simulink model "HL0905_2"  (R2018b)
settings: Solver=ode3  StartTime=0.0  StopTime=1  FixedStep=0.001  RelTol=1e-3  EnableMultiTasking=on
undefined symbols (not defined in the file): X, Y, Z
libraries: sm_lib x55, nesl_utility x11
(part 1 of 2)
settings Model: Creator=hdu  LastModifiedBy=mails
settings DataIOCC: LimitDataPoints=on  SaveFormat=Array
settings OptimizationCC: LifeSpan=inf
settings DebuggingCC: SolverPrmCheckMsg=warning  SFUnexpectedBacktrackingDiag=warning  SFNoUnconditionalDefaultTransitionDiag=warning  SFExecutionAtInitializationDiag=none
settings HardwareCC: ProdBitPerPointer=32  ProdBitPerSizeT=32  ProdBitPerPtrDiffT=32  ProdLargestAtomicFloat=None  ProdIntDivRoundTo=Undefined  ProdEndianess=Unspecified  ProdWordSize=32  ProdHWDeviceType=32-bit Generic
settings ModelReferenceCC: PropagateSignalLabelsOutOfModel=off
settings SFSimCC: SimUseLocalCustomCode=off
settings RTWCC: RTWUseLocalCustomCode=off
settings CodeAppCC: StateflowObjectComments=on
settings GRTTargetCC: TargetLangStandard=C89/C90 (ANSI)  GeneratePreprocessorConditionals=Disable all
settings ConfigComp: CovMetricSettings=dw  CovHtmlReporting=on  CovSaveCumulativeToWorkspaceVar=on  CovSaveSingleToWorkspaceVar=on  CovExternalEMLEnable=off  CovSFcnEnable=off
settings SimscapeCC: SimscapeNormalizeSystem=off
settings ConfigurationSet: Description=SimMechanics 2G

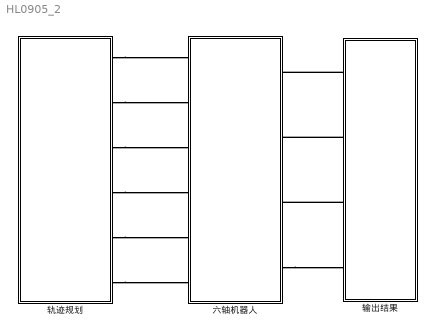
== system HL0905_2 ==
  六轴机器人 : Subsystem
  轨迹规划 : Subsystem
  输出结果 : Subsystem
  connections:
  轨迹规划/RConn1 -- 六轴机器人/LConn1
  轨迹规划/RConn2 -- 六轴机器人/LConn2
  轨迹规划/RConn3 -- 六轴机器人/LConn3
  轨迹规划/RConn4 -- 六轴机器人/LConn4
  轨迹规划/RConn6 -- 六轴机器人/LConn6
  轨迹规划/RConn5 -- 六轴机器人/LConn5
  输出结果/LConn1 -- 六轴机器人/RConn1
  输出结果/LConn2 -- 六轴机器人/RConn2
  输出结果/LConn3 -- 六轴机器人/RConn3
  六轴机器人/RConn4 -- 输出结果/LConn4

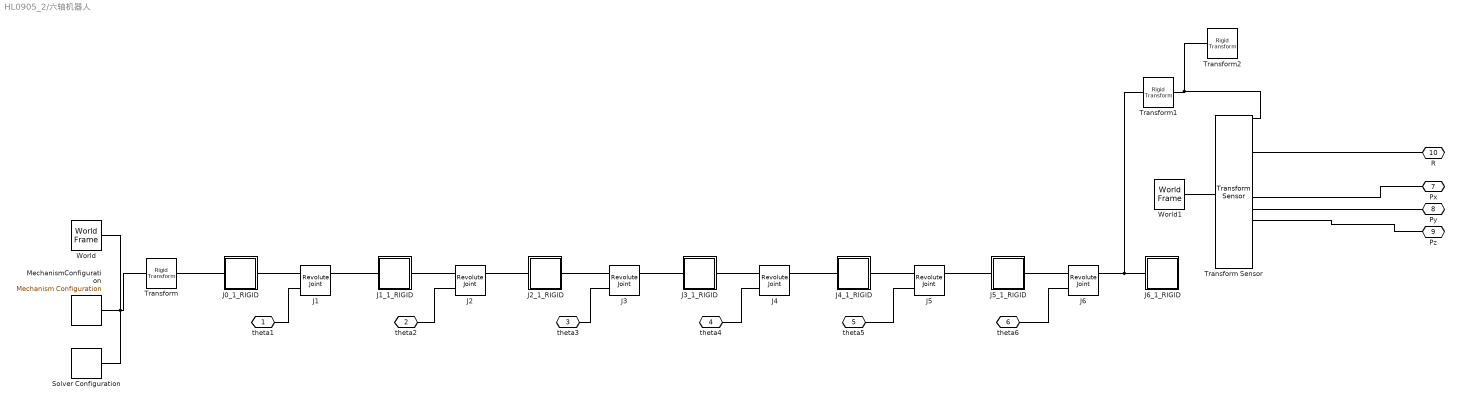
== system HL0905_2/六轴机器人 ==
  J0_1_RIGID : Subsystem
  J1 : sm_lib/Joints/Revolute Joint  SenseConstraintForce=off  SenseConstraintForceX=off  SenseConstraintForceY=off  SenseConstraintForceZ=off  SenseConstraintTorque=off  SenseConstraintTorqueX=off  SenseConstraintTorqueY=off  SenseConstraintTorqueZ=off  SenseTotalForce=off  SenseTotalForceX=off  SenseTotalForceY=off  SenseTotalForceZ=off  SenseTotalTorque=off  SenseTotalTorqueX=off  SenseTotalTorqueY=off  SenseTotalTorqueZ=off  CompositeWrenchDir=FollowerOnBase  CompositeWrenchFrame=BaseFrame  EquilibriumPosition=0  EquilibriumPositionUnits=rad  SpringStiffness=0  SpringStiffnessUnits=m*N/rad  DampingCoefficient=0  DampingCoefficientUnits=m*s*N/rad  TorqueActuationMode=ComputedTorque  MotionActuationMode=InputMotion  SensePosition=off  SenseVelocity=off  SenseAcceleration=off  SenseTorqueForce=on  PositionTargetSpecify=on  PositionTargetPriority=Low  PositionTargetValue=0  PositionTargetValueUnits=deg  VelocityTargetSpecify=off  VelocityTargetPriority=High  VelocityTargetValue=0  VelocityTargetValueUnits=deg/s
  J1_1_RIGID : Subsystem
  J2 : sm_lib/Joints/Revolute Joint  SenseConstraintForce=off  SenseConstraintForceX=off  SenseConstraintForceY=off  SenseConstraintForceZ=off  SenseConstraintTorque=off  SenseConstraintTorqueX=off  SenseConstraintTorqueY=off  SenseConstraintTorqueZ=off  SenseTotalForce=off  SenseTotalForceX=off  SenseTotalForceY=off  SenseTotalForceZ=off  SenseTotalTorque=off  SenseTotalTorqueX=off  SenseTotalTorqueY=off  SenseTotalTorqueZ=off  CompositeWrenchDir=FollowerOnBase  CompositeWrenchFrame=BaseFrame  EquilibriumPosition=0  EquilibriumPositionUnits=rad  SpringStiffness=0  SpringStiffnessUnits=m*N/rad  DampingCoefficient=0  DampingCoefficientUnits=m*s*N/rad  TorqueActuationMode=ComputedTorque  MotionActuationMode=InputMotion  SensePosition=off  SenseVelocity=off  SenseAcceleration=off  SenseTorqueForce=on  PositionTargetSpecify=on  PositionTargetPriority=Low  PositionTargetValue=-6.9319358640751347e-13  PositionTargetValueUnits=deg  VelocityTargetSpecify=off  VelocityTargetPriority=High  VelocityTargetValue=0  VelocityTargetValueUnits=deg/s
  J2_1_RIGID : Subsystem
  J3 : sm_lib/Joints/Revolute Joint  SenseConstraintForce=off  SenseConstraintForceX=off  SenseConstraintForceY=off  SenseConstraintForceZ=off  SenseConstraintTorque=off  SenseConstraintTorqueX=off  SenseConstraintTorqueY=off  SenseConstraintTorqueZ=off  SenseTotalForce=off  SenseTotalForceX=off  SenseTotalForceY=off  SenseTotalForceZ=off  SenseTotalTorque=off  SenseTotalTorqueX=off  SenseTotalTorqueY=off  SenseTotalTorqueZ=off  CompositeWrenchDir=FollowerOnBase  CompositeWrenchFrame=BaseFrame  EquilibriumPosition=0  EquilibriumPositionUnits=rad  SpringStiffness=0  SpringStiffnessUnits=m*N/rad  DampingCoefficient=0  DampingCoefficientUnits=m*s*N/rad  TorqueActuationMode=ComputedTorque  MotionActuationMode=InputMotion  SensePosition=off  SenseVelocity=off  SenseAcceleration=off  SenseTorqueForce=on  PositionTargetSpecify=on  PositionTargetPriority=Low  PositionTargetValue=-90  PositionTargetValueUnits=deg  VelocityTargetSpecify=off  VelocityTargetPriority=High  VelocityTargetValue=0  VelocityTargetValueUnits=deg/s
  J3_1_RIGID : Subsystem
  J4 : sm_lib/Joints/Revolute Joint  SenseConstraintForce=off  SenseConstraintForceX=off  SenseConstraintForceY=off  SenseConstraintForceZ=off  SenseConstraintTorque=off  SenseConstraintTorqueX=off  SenseConstraintTorqueY=off  SenseConstraintTorqueZ=off  SenseTotalForce=off  SenseTotalForceX=off  SenseTotalForceY=off  SenseTotalForceZ=off  SenseTotalTorque=off  SenseTotalTorqueX=off  SenseTotalTorqueY=off  SenseTotalTorqueZ=off  CompositeWrenchDir=FollowerOnBase  CompositeWrenchFrame=BaseFrame  EquilibriumPosition=0  EquilibriumPositionUnits=rad  SpringStiffness=0  SpringStiffnessUnits=m*N/rad  DampingCoefficient=0  DampingCoefficientUnits=m*s*N/rad  TorqueActuationMode=ComputedTorque  MotionActuationMode=InputMotion  SensePosition=off  SenseVelocity=off  SenseAcceleration=off  SenseTorqueForce=on  PositionTargetSpecify=on  PositionTargetPriority=Low  PositionTargetValue=0  PositionTargetValueUnits=deg  VelocityTargetSpecify=off  VelocityTargetPriority=High  VelocityTargetValue=0  VelocityTargetValueUnits=deg/s
  J4_1_RIGID : Subsystem
  J5 : sm_lib/Joints/Revolute Joint  SenseConstraintForce=off  SenseConstraintForceX=off  SenseConstraintForceY=off  SenseConstraintForceZ=off  SenseConstraintTorque=off  SenseConstraintTorqueX=off  SenseConstraintTorqueY=off  SenseConstraintTorqueZ=off  SenseTotalForce=off  SenseTotalForceX=off  SenseTotalForceY=off  SenseTotalForceZ=off  SenseTotalTorque=off  SenseTotalTorqueX=off  SenseTotalTorqueY=off  SenseTotalTorqueZ=off  CompositeWrenchDir=FollowerOnBase  CompositeWrenchFrame=BaseFrame  EquilibriumPosition=0  EquilibriumPositionUnits=rad  SpringStiffness=0  SpringStiffnessUnits=m*N/rad  DampingCoefficient=0  DampingCoefficientUnits=m*s*N/rad  TorqueActuationMode=ComputedTorque  MotionActuationMode=InputMotion  SensePosition=off  SenseVelocity=off  SenseAcceleration=off  SenseTorqueForce=on  PositionTargetSpecify=on  PositionTargetPriority=Low  PositionTargetValue=-4.4527765540484154e-14  PositionTargetValueUnits=deg  VelocityTargetSpecify=off  VelocityTargetPriority=High  VelocityTargetValue=0  VelocityTargetValueUnits=deg/s
  J5_1_RIGID : Subsystem
  J6 : sm_lib/Joints/Revolute Joint  SenseConstraintForce=off  SenseConstraintForceX=off  SenseConstraintForceY=off  SenseConstraintForceZ=off  SenseConstraintTorque=off  SenseConstraintTorqueX=off  SenseConstraintTorqueY=off  SenseConstraintTorqueZ=off  SenseTotalForce=off  SenseTotalForceX=off  SenseTotalForceY=off  SenseTotalForceZ=off  SenseTotalTorque=off  SenseTotalTorqueX=off  SenseTotalTorqueY=off  SenseTotalTorqueZ=off  CompositeWrenchDir=FollowerOnBase  CompositeWrenchFrame=BaseFrame  EquilibriumPosition=0  EquilibriumPositionUnits=rad  SpringStiffness=0  SpringStiffnessUnits=m*N/rad  DampingCoefficient=0  DampingCoefficientUnits=m*s*N/rad  TorqueActuationMode=ComputedTorque  MotionActuationMode=InputMotion  SensePosition=off  SenseVelocity=off  SenseAcceleration=off  SenseTorqueForce=on  PositionTargetSpecify=on  PositionTargetPriority=Low  PositionTargetValue=0  PositionTargetValueUnits=deg  VelocityTargetSpecify=off  VelocityTargetPriority=High  VelocityTargetValue=0  VelocityTargetValueUnits=deg/s
  J6_1_RIGID : Subsystem
  MechanismConfiguration : sm_lib/Utilities/Mechanism Configuration  UniformGravity=Constant  GravityVector=[0 0 -9.81]  GravityUnits=m/s^2  LinearizationDelta=0.001
  Solver Configuration : nesl_utility/Solver Configuration  PhysicalDomain=network_engine_domain  SubClassName=solver  LeftPortType=input  RightPortType=generic  Tones=[]  Harmonics=[]  SimulateNoise=off  Profile=off  UseLocalSampling=off  EnableSwitchedLinearOptims=on  FrequencyDomain=off  UseCCode=off  RelTol=0.001  AbsTol=1e-06  MinStep=1e-09  ToWorkspace=off  RevertToSquareIcSolve=off  NumHomotopyIterations=100  PhasorMode=off  PhasorModeNumHarmonics=1  DoDC=off  ResidualTolerance=1e-09  UseLocalSolver=off  LocalSolverChoice=NE_BACKWARD_EULER_ADVANCER  LocalSolverSampleTime=0.001  DoFixedCost=off  MaxNonlinIter=3  MaxModeIter=2  LinearAlgebra=Sparse  EquationFormulation=NE_TIME_EF  DelaysMemoryBudget=1024  AutomaticFiltering=on  FilteringTimeConstant=0.001  PartitionStorageMethod=AS_NEEDED  PartitionMemoryBudget=1024
  Transform : sm_lib/Frames and Transforms/Rigid Transform  TranslationMethod=Cartesian  TranslationStandardOffset=0  TranslationLengthUnit=mm  TranslationStandardAxis=+Z  TranslationCartesianOffset=[0 0 300]  TranslationROffset=0  TranslationROffsetUnits=m  TranslationZOffset=0  TranslationZOffsetUnits=m  TranslationThetaOffset=0  TranslationThetaOffsetUnits=deg  RotationMethod=ArbitraryAxis  RotationAngleUnits=rad  RotationStandardAxis=+Z  RotationAngle=1.5707963267948966  RotationArbitraryAxis=[7.8504622934188758e-17 -1.2449156633998499e-16 1]  FollAlignAxisA=+X  BaseAlignAxisA=+Y  FollAlignAxisB=+Y  BaseAlignAxisB=+Z  RotationSequenceAxes=FollowerAxes  RotationSequence=XYX  RotationSequenceAngles=[0 0 0]  RotationSequenceAnglesUnits=deg  RotationMatrix=[1 0 0; 0 1 0; 0 0 1]
  Transform Sensor : sm_lib/Frames and Transforms/Transform Sensor  MeasurementFrame=World  SenseAngle=on  SenseAxis=on  SenseAngle1=off  SenseAngle2=off  SenseAngle3=off  SenseQ=off  SenseR=on  SenseOmegaX=on  SenseOmegaY=on  SenseOmegaZ=on  SenseOmega1=off  SenseOmega2=off  SenseOmega3=off  SenseQDot=off  SenseRDot=off  SenseAlphaX=off  SenseAlphaY=off  SenseAlphaZ=off  SenseAlpha1=off  SenseAlpha2=off  SenseAlpha3=off  SenseQDDot=off  SenseRDDot=off  SenseX=on  SenseY=on  SenseZ=on  SenseRad=off  SenseAzim=off  SenseDist=off  SenseInc=off  SenseXDot=off  SenseYDot=on  SenseZDot=on  SenseRadDot=off  SenseAzimDot=off  SenseDistDot=off  SenseIncDot=off  SenseXDDot=off  SenseYDDot=on  SenseZDDot=on  SenseRadDDot=off  SenseAzimDDot=off  SenseDistDDot=off  SenseIncDDot=off
  Transform1 : sm_lib/Frames and Transforms/Rigid Transform  TranslationMethod=Cartesian  TranslationStandardOffset=0  TranslationLengthUnit=mm  TranslationStandardAxis=+X  TranslationCartesianOffset=[0 0 151.194984090458]  TranslationROffset=0  TranslationROffsetUnits=m  TranslationZOffset=0  TranslationZOffsetUnits=m  TranslationThetaOffset=0  TranslationThetaOffsetUnits=deg  RotationMethod=None  RotationAngleUnits=rad  RotationStandardAxis=+Z  RotationAngle=3.1415926535897931  RotationArbitraryAxis=[0 5.5511151231257827e-17 -1]  FollAlignAxisA=+X  BaseAlignAxisA=+Y  FollAlignAxisB=+Y  BaseAlignAxisB=+Z  RotationSequenceAxes=FollowerAxes  RotationSequence=XYX  RotationSequenceAngles=[0 0 0]  RotationSequenceAnglesUnits=deg  RotationMatrix=[1 0 0; 0 1 0; 0 0 1]
  Transform2 : sm_lib/Frames and Transforms/Rigid Transform  TranslationMethod=Cartesian  TranslationStandardOffset=0  TranslationLengthUnit=mm  TranslationStandardAxis=+X  TranslationCartesianOffset=[0 0 124.08]  TranslationROffset=0  TranslationROffsetUnits=m  TranslationZOffset=0  TranslationZOffsetUnits=m  TranslationThetaOffset=0  TranslationThetaOffsetUnits=deg  RotationMethod=None  RotationAngleUnits=rad  RotationStandardAxis=+Z  RotationAngle=3.1415926535897931  RotationArbitraryAxis=[0 5.5511151231257827e-17 -1]  FollAlignAxisA=+X  BaseAlignAxisA=+Y  FollAlignAxisB=+Y  BaseAlignAxisB=+Z  RotationSequenceAxes=FollowerAxes  RotationSequence=XYX  RotationSequenceAngles=[0 0 0]  RotationSequenceAnglesUnits=deg  RotationMatrix=[1 0 0; 0 1 0; 0 0 1]
  World : sm_lib/Frames and Transforms/World Frame
  World1 : sm_lib/Frames and Transforms/World Frame
  theta1 : PMIOPort  Side=Left
  theta2 : PMIOPort  Port=2  Side=Left
  theta3 : PMIOPort  Port=3  Side=Left
  theta4 : PMIOPort  Port=4  Side=Left
  theta5 : PMIOPort  Port=5  Side=Left
  theta6 : PMIOPort  Port=6  Side=Left
  Px : PMIOPort  Port=7  Side=Right
  Py : PMIOPort  Port=8  Side=Right
  Pz : PMIOPort  Port=9  Side=Right
  R : PMIOPort  Port=10  Side=Right
  connections:
  theta3/RConn1 -- J3/LConn2
  theta5/RConn1 -- J5/LConn2
  J0_1_RIGID/LConn1 -- Transform/RConn1
  J4_1_RIGID/LConn1 -- J4/RConn1
  J1_1_RIGID/RConn1 -- J2/LConn1
  J1_1_RIGID/LConn1 -- J1/RConn1
  J6_1_RIGID/LConn1 -- Transform1/LConn1 -- J6/RConn1
  J4_1_RIGID/RConn1 -- J5/LConn1
  J5_1_RIGID/RConn1 -- J6/LConn1
  J2_1_RIGID/LConn1 -- J2/RConn1
  J3_1_RIGID/RConn1 -- J4/LConn1
  J3_1_RIGID/LConn1 -- J3/RConn1
  theta2/RConn1 -- J2/LConn2
  theta6/RConn1 -- J6/LConn2
  theta1/RConn1 -- J1/LConn2
  Transform/LConn1 -- MechanismConfiguration/RConn1 -- Solver Configuration/RConn1 -- World/RConn1
  J0_1_RIGID/RConn1 -- J1/LConn1
  J2_1_RIGID/RConn1 -- J3/LConn1
  J5_1_RIGID/LConn1 -- J5/RConn1
  theta4/RConn1 -- J4/LConn2
  World1/RConn1 -- Transform Sensor/LConn1
  Transform Sensor/RConn8 -- Px/RConn1
  Pz/RConn1 -- Transform Sensor/RConn10
  Transform1/RConn1 -- Transform Sensor/RConn1 -- Transform2/LConn1
  Py/RConn1 -- Transform Sensor/RConn9
  R/RConn1 -- Transform Sensor/RConn4

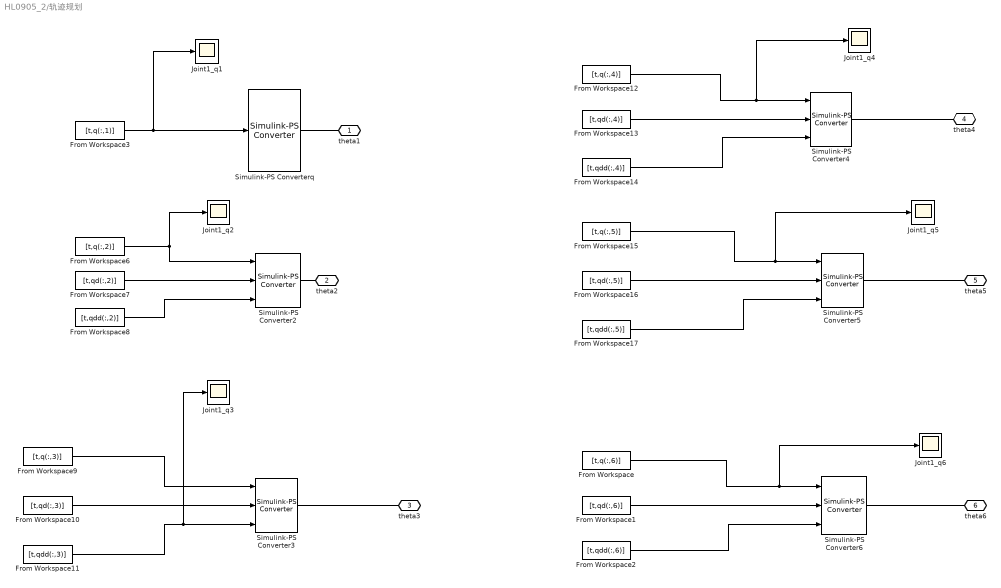
== system HL0905_2/轨迹规划 ==
  From Workspace : FromWorkspace  VariableName=[t,q(:,6)]  SampleTime=0
  From Workspace1 : FromWorkspace  VariableName=[t,qd(:,6)]  SampleTime=0
  From Workspace10 : FromWorkspace  VariableName=[t,qd(:,3)]  SampleTime=0
  From Workspace11 : FromWorkspace  VariableName=[t,qdd(:,3)]  SampleTime=0
  From Workspace12 : FromWorkspace  VariableName=[t,q(:,4)]  SampleTime=0
  From Workspace13 : FromWorkspace  VariableName=[t,qd(:,4)]  SampleTime=0
  From Workspace14 : FromWorkspace  VariableName=[t,qdd(:,4)]  SampleTime=0
  From Workspace15 : FromWorkspace  VariableName=[t,q(:,5)]  SampleTime=0
  From Workspace16 : FromWorkspace  VariableName=[t,qd(:,5)]  SampleTime=0
  From Workspace17 : FromWorkspace  VariableName=[t,qdd(:,5)]  SampleTime=0
  From Workspace2 : FromWorkspace  VariableName=[t,qdd(:,6)]  SampleTime=0
  From Workspace3 : FromWorkspace  VariableName=[t,q(:,1)]  SampleTime=0
  From Workspace6 : FromWorkspace  VariableName=[t,q(:,2)]  SampleTime=0
  From Workspace7 : FromWorkspace  VariableName=[t,qd(:,2)]  SampleTime=0
  From Workspace8 : FromWorkspace  VariableName=[t,qdd(:,2)]  SampleTime=0
  From Workspace9 : FromWorkspace  VariableName=[t,q(:,3)]  SampleTime=0
  Joint1_q{1..6} (6 alike) : Scope
  Simulink-PS Converter{2..6} (5 alike) : nesl_utility/Simulink-PS Converter  PhysicalDomain=network_engine_domain  SubClassName=ps_input  LeftPortType=input  RightPortType=output  PseudoPeriodic=off  Frequencies=[]  NoiseDistribution=none  NoiseParameters=[]  Unit=rad  AffineConversion=off  FilteringAndDerivatives=provide  SimscapeFilterOrder=2  InputFilterTimeConstant=0.01  UdotUserProvided=2
  Simulink-PS Converterq : nesl_utility/Simulink-PS Converter  PhysicalDomain=network_engine_domain  SubClassName=ps_input  LeftPortType=input  RightPortType=output  PseudoPeriodic=off  Frequencies=[]  NoiseDistribution=none  NoiseParameters=[]  Unit=rad  AffineConversion=off  FilteringAndDerivatives=provide  SimscapeFilterOrder=2  InputFilterTimeConstant=0.01  UdotUserProvided=0
  theta1 : PMIOPort  Side=Right
  theta2 : PMIOPort  Port=2  Side=Right
  theta3 : PMIOPort  Port=3  Side=Right
  theta4 : PMIOPort  Port=4  Side=Right
  theta5 : PMIOPort  Port=5  Side=Right
  theta6 : PMIOPort  Port=6  Side=Right
  wires:
  From Workspace1/1 -> Simulink-PS Converter6/2
  From Workspace2/1 -> Simulink-PS Converter6/3
  From Workspace/1 -> Joint1_q6/1, Simulink-PS Converter6/1
  From Workspace3/1 -> Joint1_q1/1, Simulink-PS Converterq/1
  From Workspace7/1 -> Simulink-PS Converter2/2
  From Workspace8/1 -> Simulink-PS Converter2/3
  From Workspace6/1 -> Simulink-PS Converter2/1, Joint1_q2/1
  From Workspace10/1 -> Simulink-PS Converter3/2
  From Workspace11/1 -> Joint1_q3/1, Simulink-PS Converter3/3
  From Workspace9/1 -> Simulink-PS Converter3/1
  From Workspace13/1 -> Simulink-PS Converter4/2
  From Workspace14/1 -> Simulink-PS Converter4/3
  From Workspace12/1 -> Joint1_q4/1, Simulink-PS Converter4/1
  From Workspace16/1 -> Simulink-PS Converter5/2
  From Workspace17/1 -> Simulink-PS Converter5/3
  From Workspace15/1 -> Joint1_q5/1, Simulink-PS Converter5/1
  connections:
  Simulink-PS Converterq/RConn1 -- theta1/RConn1
  Simulink-PS Converter2/RConn1 -- theta2/RConn1
  Simulink-PS Converter3/RConn1 -- theta3/RConn1
  Simulink-PS Converter4/RConn1 -- theta4/RConn1
  Simulink-PS Converter5/RConn1 -- theta5/RConn1
  theta6/RConn1 -- Simulink-PS Converter6/RConn1

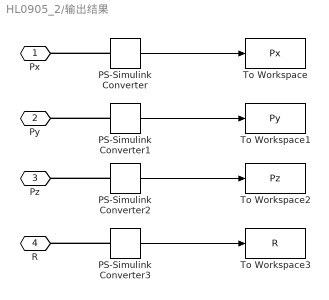
== system HL0905_2/输出结果 ==
  PS-Simulink Converter : nesl_utility/PS-Simulink Converter  PhysicalDomain=network_engine_domain  SubClassName=ps_output  LeftPortType=input  RightPortType=output  PseudoPeriodic=off  Frequencies=[]  Unit=mm  AffineConversion=off
  PS-Simulink Converter1 : nesl_utility/PS-Simulink Converter  PhysicalDomain=network_engine_domain  SubClassName=ps_output  LeftPortType=input  RightPortType=output  PseudoPeriodic=off  Frequencies=[]  Unit=mm  AffineConversion=off
  PS-Simulink Converter2 : nesl_utility/PS-Simulink Converter  PhysicalDomain=network_engine_domain  SubClassName=ps_output  LeftPortType=input  RightPortType=output  PseudoPeriodic=off  Frequencies=[]  Unit=mm  AffineConversion=off
  PS-Simulink Converter3 : nesl_utility/PS-Simulink Converter  PhysicalDomain=network_engine_domain  SubClassName=ps_output  LeftPortType=input  RightPortType=output  PseudoPeriodic=off  Frequencies=[]  Unit=1  AffineConversion=off
  To Workspace : ToWorkspace  VariableName=Px  SampleTime=-1
      settings: Save2DSignal=2-D array (concatenate along first dimension)
  To Workspace1 : ToWorkspace  VariableName=Py  SampleTime=-1
      settings: Save2DSignal=2-D array (concatenate along first dimension)
  To Workspace2 : ToWorkspace  VariableName=Pz  SampleTime=-1
      settings: Save2DSignal=2-D array (concatenate along first dimension)
  To Workspace3 : ToWorkspace  VariableName=R  SampleTime=-1
      settings: Save2DSignal=2-D array (concatenate along first dimension)
  Px : PMIOPort  Side=Left
  Py : PMIOPort  Port=2  Side=Left
  Pz : PMIOPort  Port=3  Side=Left
  R : PMIOPort  Port=4  Side=Left
  wires:
  PS-Simulink Converter/1 -> To Workspace/1
  PS-Simulink Converter1/1 -> To Workspace1/1
  PS-Simulink Converter2/1 -> To Workspace2/1
  PS-Simulink Converter3/1 -> To Workspace3/1
  connections:
  PS-Simulink Converter1/LConn1 -- Py/RConn1
  PS-Simulink Converter/LConn1 -- Px/RConn1
  PS-Simulink Converter2/LConn1 -- Pz/RConn1
  PS-Simulink Converter3/LConn1 -- R/RConn1

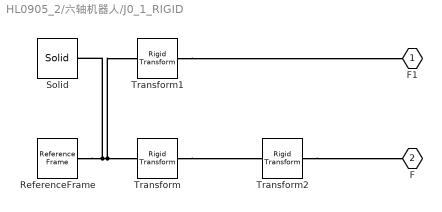
== system HL0905_2/六轴机器人/J0_1_RIGID ==
  ReferenceFrame : sm_lib/Frames and Transforms/Reference Frame
  Solid : sm_lib/Body Elements/Solid  InertiaType=Custom  Mass=7.6540594351842266  MassUnits=kg  CenterOfMass=[22.860239072093147 -147.21867176219041 -1.2431125209809186]  CenterOfMassUnits=mm  MomentsOfInertia=[130694.70688402398 123509.99199142594 133535.69433842544]  MomentsOfInertiaUnits=kg*mm^2  ProductsOfInertia=[-1577.6165993481045 1190.9909643824089 5823.7333434025841]  ProductsOfInertiaUnits=kg*mm^2  BasedOnType=Density  Density=1000  DensityUnits=kg/(m^3)  DoExposeReferenceFrame=on  SerializedFrames=<Frames/>  GraphicType=FromGeometry  MarkerShape=Sphere  MarkerSize=10  MarkerSizeUnits=m  GraphicVisPropType=SimpleVisualProperties  GraphicDiffuseColor=[0.2 0.2 0.2]  GraphicSpecularColor=[0.5 0.5 0.5 1.0]  GraphicAmbientColor=[0.15 0.15 0.15 1.0]  GraphicEmissiveColor=[0.0 0.0 0.0 1.0]  GraphicShininess=75  GraphicOpacity=1  GeometryShape=FromFile  RectangleSize=[1 1]  RectangleSizeUnits=m  BrickDimensions=[1 1 1]  BrickDimensionUnits=m  CylinderRadius=1  CylinderRadiusUnits=m  CylinderLength=1  CylinderLengthUnits=m  SphereRadius=1  SphereRadiusUnits=m  EllipsoidRadii=[1 1 1]  EllipsoidRadiiUnits=m  ExtrusionCrossSection=[1 1; -1 1; -1 -1; 1 -1]  ExtrusionCrossSectionUnits=m  ExtrusionLength=1  ExtrusionLengthUnits=m  PolygonNumSides=3  PolygonOuterRadius=1  PolygonOuterRadiusUnits=m  ExtGeomFileType=STL  ExtGeomFileName=J0_默认_sldprt.STL  ExtGeomFileUnits=mm  RevolutionCrossSection=[1 1; 1 -1; 2 -1; 2 1]  RevolutionCrossSectionUnits=m  RevolutionExtent=Full  RevolutionAngle=180  RevolutionAngleUnits=deg
  Transform : sm_lib/Frames and Transforms/Rigid Transform  TranslationMethod=Cartesian  TranslationStandardOffset=0  TranslationLengthUnit=mm  TranslationStandardAxis=+Z  TranslationCartesianOffset=[-1.1006414838582221e-13 -330.45657177129794 1.4155343563970754e-12]  TranslationROffset=0  TranslationROffsetUnits=m  TranslationZOffset=0  TranslationZOffsetUnits=m  TranslationThetaOffset=0  TranslationThetaOffsetUnits=deg  RotationMethod=ArbitraryAxis  RotationAngleUnits=rad  RotationStandardAxis=+Z  RotationAngle=2.0943951023931957  RotationArbitraryAxis=[-0.57735026918962584 -0.57735026918962562 -0.57735026918962584]  FollAlignAxisA=+X  BaseAlignAxisA=+Y  FollAlignAxisB=+Y  BaseAlignAxisB=+Z  RotationSequenceAxes=FollowerAxes  RotationSequence=XYX  RotationSequenceAngles=[0 0 0]  RotationSequenceAnglesUnits=deg  RotationMatrix=[1 0 0; 0 1 0; 0 0 1]
  Transform1 : sm_lib/Frames and Transforms/Rigid Transform  TranslationMethod=Cartesian  TranslationStandardOffset=0  TranslationLengthUnit=mm  TranslationStandardAxis=+Z  TranslationCartesianOffset=[0 0 0]  TranslationROffset=0  TranslationROffsetUnits=m  TranslationZOffset=0  TranslationZOffsetUnits=m  TranslationThetaOffset=0  TranslationThetaOffsetUnits=deg  RotationMethod=ArbitraryAxis  RotationAngleUnits=rad  RotationStandardAxis=+Z  RotationAngle=2.0943951023931957  RotationArbitraryAxis=[-0.57735026918962584 -0.57735026918962562 -0.57735026918962584]  FollAlignAxisA=+X  BaseAlignAxisA=+Y  FollAlignAxisB=+Y  BaseAlignAxisB=+Z  RotationSequenceAxes=FollowerAxes  RotationSequence=XYX  RotationSequenceAngles=[0 0 0]  RotationSequenceAnglesUnits=deg  RotationMatrix=[1 0 0; 0 1 0; 0 0 1]
  Transform2 : sm_lib/Frames and Transforms/Rigid Transform  TranslationMethod=Cartesian  TranslationStandardOffset=0  TranslationLengthUnit=mm  TranslationStandardAxis=+Z  TranslationCartesianOffset=[0 0 0]  TranslationROffset=0  TranslationROffsetUnits=m  TranslationZOffset=0  TranslationZOffsetUnits=m  TranslationThetaOffset=0  TranslationThetaOffsetUnits=deg  RotationMethod=StandardAxis  RotationAngleUnits=deg  RotationStandardAxis=+Z  RotationAngle=-90  RotationArbitraryAxis=[-0.57735026918962584 -0.57735026918962562 -0.57735026918962584]  FollAlignAxisA=+X  BaseAlignAxisA=+Y  FollAlignAxisB=+Y  BaseAlignAxisB=+Z  RotationSequenceAxes=FollowerAxes  RotationSequence=XYX  RotationSequenceAngles=[0 0 0]  RotationSequenceAnglesUnits=deg  RotationMatrix=[1 0 0; 0 1 0; 0 0 1]
  F1 : PMIOPort  Side=Left
  F : PMIOPort  Port=2  Side=Right
  connections:
  Solid/RConn1 -- ReferenceFrame/RConn1 -- Transform/LConn1 -- Transform1/LConn1
  Transform/RConn1 -- Transform2/LConn1
  Transform2/RConn1 -- F/RConn1
  Transform1/RConn1 -- F1/RConn1

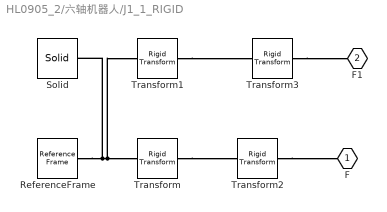
== system HL0905_2/六轴机器人/J1_1_RIGID ==
  ReferenceFrame : sm_lib/Frames and Transforms/Reference Frame
  Solid : sm_lib/Body Elements/Solid  InertiaType=Custom  Mass=10.630000000000001  MassUnits=kg  CenterOfMass=[38.979999999999997 5.6399999999999997 -87]  CenterOfMassUnits=mm  MomentsOfInertia=[58730.529999999999 75050.639999999999 55241.57]  MomentsOfInertiaUnits=kg*mm^2  ProductsOfInertia=[-528.18999999999994 -10070.20999999999 -853.15999999999997]  ProductsOfInertiaUnits=kg*mm^2  BasedOnType=Density  Density=1000  DensityUnits=kg/(m^3)  DoExposeReferenceFrame=on  SerializedFrames=<Frames/>  GraphicType=FromGeometry  MarkerShape=Sphere  MarkerSize=10  MarkerSizeUnits=m  GraphicVisPropType=SimpleVisualProperties  GraphicDiffuseColor=[1 1 1]  GraphicSpecularColor=[0.5 0.5 0.5 1.0]  GraphicAmbientColor=[0.15 0.15 0.15 1.0]  GraphicEmissiveColor=[0.0 0.0 0.0 1.0]  GraphicShininess=75  GraphicOpacity=1  GeometryShape=FromFile  RectangleSize=[1 1]  RectangleSizeUnits=m  BrickDimensions=[1 1 1]  BrickDimensionUnits=m  CylinderRadius=1  CylinderRadiusUnits=m  CylinderLength=1  CylinderLengthUnits=m  SphereRadius=1  SphereRadiusUnits=m  EllipsoidRadii=[1 1 1]  EllipsoidRadiiUnits=m  ExtrusionCrossSection=[1 1; -1 1; -1 -1; 1 -1]  ExtrusionCrossSectionUnits=m  ExtrusionLength=1  ExtrusionLengthUnits=m  PolygonNumSides=3  PolygonOuterRadius=1  PolygonOuterRadiusUnits=m  ExtGeomFileType=STL  ExtGeomFileName=J1_默认_sldprt.STL  ExtGeomFileUnits=mm  RevolutionCrossSection=[1 1; 1 -1; 2 -1; 2 1]  RevolutionCrossSectionUnits=m  RevolutionExtent=Full  RevolutionAngle=180  RevolutionAngleUnits=deg
  Transform : sm_lib/Frames and Transforms/Rigid Transform  TranslationMethod=Cartesian  TranslationStandardOffset=0  TranslationLengthUnit=mm  TranslationStandardAxis=+Z  TranslationCartesianOffset=[-1.5175638523601265e-12 0.46986063114494953 -521.58681036714142]  TranslationROffset=0  TranslationROffsetUnits=m  TranslationZOffset=0  TranslationZOffsetUnits=m  TranslationThetaOffset=0  TranslationThetaOffsetUnits=deg  RotationMethod=ArbitraryAxis  RotationAngleUnits=rad  RotationStandardAxis=+Z  RotationAngle=4.6857050202360969e-15  RotationArbitraryAxis=[0.043683951669101606 0.99904540055323376 1.0224735728616534e-16]  FollAlignAxisA=+X  BaseAlignAxisA=+Y  FollAlignAxisB=+Y  BaseAlignAxisB=+Z  RotationSequenceAxes=FollowerAxes  RotationSequence=XYX  RotationSequenceAngles=[0 0 0]  RotationSequenceAnglesUnits=deg  RotationMatrix=[1 0 0; 0 1 0; 0 0 1]
  Transform1 : sm_lib/Frames and Transforms/Rigid Transform  TranslationMethod=Cartesian  TranslationStandardOffset=0  TranslationLengthUnit=mm  TranslationStandardAxis=+Z  TranslationCartesianOffset=[-157.5018651542409 0.46986063114702603 -0.13023859582908526]  TranslationROffset=0  TranslationROffsetUnits=m  TranslationZOffset=0  TranslationZOffsetUnits=m  TranslationThetaOffset=0  TranslationThetaOffsetUnits=deg  RotationMethod=ArbitraryAxis  RotationAngleUnits=rad  RotationStandardAxis=+Z  RotationAngle=2.0943951023932077  RotationArbitraryAxis=[0.57735026918961752 0.57735026918962995 0.57735026918962984]  FollAlignAxisA=+X  BaseAlignAxisA=+Y  FollAlignAxisB=+Y  BaseAlignAxisB=+Z  RotationSequenceAxes=FollowerAxes  RotationSequence=XYX  RotationSequenceAngles=[0 0 0]  RotationSequenceAnglesUnits=deg  RotationMatrix=[1 0 0; 0 1 0; 0 0 1]
  Transform2 : sm_lib/Frames and Transforms/Rigid Transform  TranslationMethod=Cartesian  TranslationStandardOffset=0  TranslationLengthUnit=mm  TranslationStandardAxis=+Z  TranslationCartesianOffset=[0 0 0]  TranslationROffset=0  TranslationROffsetUnits=m  TranslationZOffset=0  TranslationZOffsetUnits=m  TranslationThetaOffset=0  TranslationThetaOffsetUnits=deg  RotationMethod=StandardAxis  RotationAngleUnits=deg  RotationStandardAxis=+Z  RotationAngle=90  RotationArbitraryAxis=[-0.57735026918962584 -0.57735026918962562 -0.57735026918962584]  FollAlignAxisA=+X  BaseAlignAxisA=+Y  FollAlignAxisB=+Y  BaseAlignAxisB=+Z  RotationSequenceAxes=FollowerAxes  RotationSequence=XYX  RotationSequenceAngles=[0 0 0]  RotationSequenceAnglesUnits=deg  RotationMatrix=[1 0 0; 0 1 0; 0 0 1]
  Transform3 : sm_lib/Frames and Transforms/Rigid Transform  TranslationMethod=Cartesian  TranslationStandardOffset=0  TranslationLengthUnit=mm  TranslationStandardAxis=+Z  TranslationCartesianOffset=[0 0 0]  TranslationROffset=0  TranslationROffsetUnits=m  TranslationZOffset=0  TranslationZOffsetUnits=m  TranslationThetaOffset=0  TranslationThetaOffsetUnits=deg  RotationMethod=AlignedAxes  RotationAngleUnits=deg  RotationStandardAxis=+Z  RotationAngle=90  RotationArbitraryAxis=[-0.57735026918962584 -0.57735026918962562 -0.57735026918962584]  FollAlignAxisA=+Z  BaseAlignAxisA=-Z  FollAlignAxisB=+Y  BaseAlignAxisB=+X  RotationSequenceAxes=FollowerAxes  RotationSequence=XYX  RotationSequenceAngles=[0 0 0]  RotationSequenceAnglesUnits=deg  RotationMatrix=[1 0 0; 0 1 0; 0 0 1]
  F : PMIOPort  Side=Left
  F1 : PMIOPort  Port=2  Side=Right
  connections:
  Solid/RConn1 -- ReferenceFrame/RConn1 -- Transform/LConn1 -- Transform1/LConn1
  Transform2/RConn1 -- F/RConn1
  Transform3/RConn1 -- F1/RConn1
  Transform/RConn1 -- Transform2/LConn1
  Transform1/RConn1 -- Transform3/LConn1

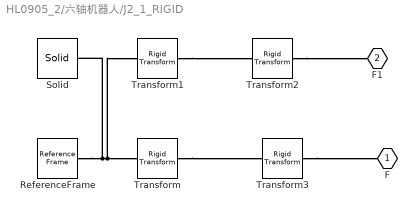
== system HL0905_2/六轴机器人/J2_1_RIGID ==
  ReferenceFrame : sm_lib/Frames and Transforms/Reference Frame
  Solid : sm_lib/Body Elements/Solid  InertiaType=Custom  Mass=13.369999999999999  MassUnits=kg  CenterOfMass=[-9.3499999999999996 -290.32999999999998 13.24]  CenterOfMassUnits=mm  MomentsOfInertia=[305534.1999999999 54660.519999999997 294009.64000000001]  MomentsOfInertiaUnits=kg*mm^2  ProductsOfInertia=[5354.0299999999979 -968.77999999999997 5458.8599999999997]  ProductsOfInertiaUnits=kg*mm^2  BasedOnType=Density  Density=1000  DensityUnits=kg/(m^3)  DoExposeReferenceFrame=on  SerializedFrames=<Frames/>  GraphicType=FromGeometry  MarkerShape=Sphere  MarkerSize=10  MarkerSizeUnits=m  GraphicVisPropType=SimpleVisualProperties  GraphicDiffuseColor=[1 1 1]  GraphicSpecularColor=[0.5 0.5 0.5 1.0]  GraphicAmbientColor=[0.15 0.15 0.15 1.0]  GraphicEmissiveColor=[0.0 0.0 0.0 1.0]  GraphicShininess=75  GraphicOpacity=1  GeometryShape=FromFile  RectangleSize=[1 1]  RectangleSizeUnits=m  BrickDimensions=[1 1 1]  BrickDimensionUnits=m  CylinderRadius=1  CylinderRadiusUnits=m  CylinderLength=1  CylinderLengthUnits=m  SphereRadius=1  SphereRadiusUnits=m  EllipsoidRadii=[1 1 1]  EllipsoidRadiiUnits=m  ExtrusionCrossSection=[1 1; -1 1; -1 -1; 1 -1]  ExtrusionCrossSectionUnits=m  ExtrusionLength=1  ExtrusionLengthUnits=m  PolygonNumSides=3  PolygonOuterRadius=1  PolygonOuterRadiusUnits=m  ExtGeomFileType=STL  ExtGeomFileName=J2_默认_sldprt.STL  ExtGeomFileUnits=mm  RevolutionCrossSection=[1 1; 1 -1; 2 -1; 2 1]  RevolutionCrossSectionUnits=m  RevolutionExtent=Full  RevolutionAngle=180  RevolutionAngleUnits=deg
  Transform : sm_lib/Frames and Transforms/Rigid Transform  TranslationMethod=Cartesian  TranslationStandardOffset=0  TranslationLengthUnit=mm  TranslationStandardAxis=+Z  TranslationCartesianOffset=[-1.1161902030621819e-12 -450.00000000000068 -157.50186515424167]  TranslationROffset=0  TranslationROffsetUnits=m  TranslationZOffset=0  TranslationZOffsetUnits=m  TranslationThetaOffset=0  TranslationThetaOffsetUnits=deg  RotationMethod=ArbitraryAxis  RotationAngleUnits=rad  RotationStandardAxis=+Z  RotationAngle=2.2022005471504983e-14  RotationArbitraryAxis=[-0.2016570245724037 0.97945619832670661 -2.1748296459883953e-15]  FollAlignAxisA=+X  BaseAlignAxisA=+Y  FollAlignAxisB=+Y  BaseAlignAxisB=+Z  RotationSequenceAxes=FollowerAxes  RotationSequence=XYX  RotationSequenceAngles=[0 0 0]  RotationSequenceAnglesUnits=deg  RotationMatrix=[1 0 0; 0 1 0; 0 0 1]
  Transform1 : sm_lib/Frames and Transforms/Rigid Transform  TranslationMethod=Cartesian  TranslationStandardOffset=0  TranslationLengthUnit=mm  TranslationStandardAxis=+Z  TranslationCartesianOffset=[0 0 -249.10747383836633]  TranslationROffset=0  TranslationROffsetUnits=m  TranslationZOffset=0  TranslationZOffsetUnits=m  TranslationThetaOffset=0  TranslationThetaOffsetUnits=deg  RotationMethod=ArbitraryAxis  RotationAngleUnits=rad  RotationStandardAxis=+Z  RotationAngle=0  RotationArbitraryAxis=[0 0 0]  FollAlignAxisA=+X  BaseAlignAxisA=+Y  FollAlignAxisB=+Y  BaseAlignAxisB=+Z  RotationSequenceAxes=FollowerAxes  RotationSequence=XYX  RotationSequenceAngles=[0 0 0]  RotationSequenceAnglesUnits=deg  RotationMatrix=[1 0 0; 0 1 0; 0 0 1]
  Transform2 : sm_lib/Frames and Transforms/Rigid Transform  TranslationMethod=Cartesian  TranslationStandardOffset=0  TranslationLengthUnit=mm  TranslationStandardAxis=+Z  TranslationCartesianOffset=[0 0 0]  TranslationROffset=0  TranslationROffsetUnits=m  TranslationZOffset=0  TranslationZOffsetUnits=m  TranslationThetaOffset=0  TranslationThetaOffsetUnits=deg  RotationMethod=AlignedAxes  RotationAngleUnits=deg  RotationStandardAxis=+Z  RotationAngle=90  RotationArbitraryAxis=[-0.57735026918962584 -0.57735026918962562 -0.57735026918962584]  FollAlignAxisA=+Z  BaseAlignAxisA=-Z  FollAlignAxisB=+Y  BaseAlignAxisB=+X  RotationSequenceAxes=FollowerAxes  RotationSequence=XYX  RotationSequenceAngles=[0 0 0]  RotationSequenceAnglesUnits=deg  RotationMatrix=[1 0 0; 0 1 0; 0 0 1]
  Transform3 : sm_lib/Frames and Transforms/Rigid Transform  TranslationMethod=Cartesian  TranslationStandardOffset=0  TranslationLengthUnit=mm  TranslationStandardAxis=+Z  TranslationCartesianOffset=[0 0 0]  TranslationROffset=0  TranslationROffsetUnits=m  TranslationZOffset=0  TranslationZOffsetUnits=m  TranslationThetaOffset=0  TranslationThetaOffsetUnits=deg  RotationMethod=AlignedAxes  RotationAngleUnits=deg  RotationStandardAxis=+Z  RotationAngle=90  RotationArbitraryAxis=[-0.57735026918962584 -0.57735026918962562 -0.57735026918962584]  FollAlignAxisA=+Z  BaseAlignAxisA=-Z  FollAlignAxisB=+Y  BaseAlignAxisB=+X  RotationSequenceAxes=FollowerAxes  RotationSequence=XYX  RotationSequenceAngles=[0 0 0]  RotationSequenceAnglesUnits=deg  RotationMatrix=[1 0 0; 0 1 0; 0 0 1]
  F : PMIOPort  Side=Left
  F1 : PMIOPort  Port=2  Side=Right
  connections:
  Solid/RConn1 -- ReferenceFrame/RConn1 -- Transform/LConn1 -- Transform1/LConn1
  Transform3/RConn1 -- F/RConn1
  Transform2/RConn1 -- F1/RConn1
  Transform/RConn1 -- Transform3/LConn1
  Transform1/RConn1 -- Transform2/LConn1

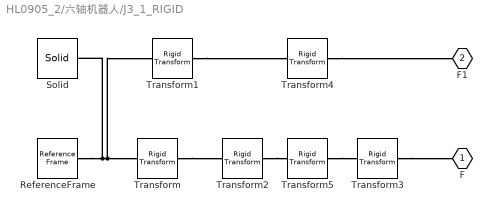
== system HL0905_2/六轴机器人/J3_1_RIGID ==
  ReferenceFrame : sm_lib/Frames and Transforms/Reference Frame
  Solid : sm_lib/Body Elements/Solid  InertiaType=Custom  Mass=5.2930000000000001  MassUnits=kg  CenterOfMass=[82.347999999999999 -6.7000000000000002 -16.399999999999999]  CenterOfMassUnits=mm  MomentsOfInertia=[9712.7630000000008 14300.983 15335.696]  MomentsOfInertiaUnits=kg*mm^2  ProductsOfInertia=[137.73699999999999 1087.2009999999993 296.08499999999998]  ProductsOfInertiaUnits=kg*mm^2  BasedOnType=Density  Density=1000  DensityUnits=kg/(m^3)  DoExposeReferenceFrame=on  SerializedFrames=<Frames/>  GraphicType=FromGeometry  MarkerShape=Sphere  MarkerSize=10  MarkerSizeUnits=m  GraphicVisPropType=SimpleVisualProperties  GraphicDiffuseColor=[1 1 1]  GraphicSpecularColor=[0.5 0.5 0.5 1.0]  GraphicAmbientColor=[0.15 0.15 0.15 1.0]  GraphicEmissiveColor=[0.0 0.0 0.0 1.0]  GraphicShininess=75  GraphicOpacity=1  GeometryShape=FromFile  RectangleSize=[1 1]  RectangleSizeUnits=m  BrickDimensions=[1 1 1]  BrickDimensionUnits=m  CylinderRadius=1  CylinderRadiusUnits=m  CylinderLength=1  CylinderLengthUnits=m  SphereRadius=1  SphereRadiusUnits=m  EllipsoidRadii=[1 1 1]  EllipsoidRadiiUnits=m  ExtrusionCrossSection=[1 1; -1 1; -1 -1; 1 -1]  ExtrusionCrossSectionUnits=m  ExtrusionLength=1  ExtrusionLengthUnits=m  PolygonNumSides=3  PolygonOuterRadius=1  PolygonOuterRadiusUnits=m  ExtGeomFileType=STL  ExtGeomFileName=J3_默认_sldprt.STL  ExtGeomFileUnits=mm  RevolutionCrossSection=[1 1; 1 -1; 2 -1; 2 1]  RevolutionCrossSectionUnits=m  RevolutionExtent=Full  RevolutionAngle=180  RevolutionAngleUnits=deg
  Transform : sm_lib/Frames and Transforms/Rigid Transform  TranslationMethod=Cartesian  TranslationStandardOffset=0  TranslationLengthUnit=mm  TranslationStandardAxis=+Z  TranslationCartesianOffset=[80.000000000010388 -1.3557155398302712e-11 249.10747383836627]  TranslationROffset=0  TranslationROffsetUnits=m  TranslationZOffset=0  TranslationZOffsetUnits=m  TranslationThetaOffset=0  TranslationThetaOffsetUnits=deg  RotationMethod=ArbitraryAxis  RotationAngleUnits=rad  RotationStandardAxis=+Z  RotationAngle=3.1415926535897931  RotationArbitraryAxis=[1 -3.7970713377376732e-47 -7.7524554575046664e-17]  FollAlignAxisA=+X  BaseAlignAxisA=+Y  FollAlignAxisB=+Y  BaseAlignAxisB=+Z  RotationSequenceAxes=FollowerAxes  RotationSequence=XYX  RotationSequenceAngles=[0 0 0]  RotationSequenceAnglesUnits=deg  RotationMatrix=[1 0 0; 0 1 0; 0 0 1]
  Transform1 : sm_lib/Frames and Transforms/Rigid Transform  TranslationMethod=Cartesian  TranslationStandardOffset=0  TranslationLengthUnit=mm  TranslationStandardAxis=+Z  TranslationCartesianOffset=[-61.209572476958321 1.1102230246251565e-13 0]  TranslationROffset=0  TranslationROffsetUnits=m  TranslationZOffset=0  TranslationZOffsetUnits=m  TranslationThetaOffset=0  TranslationThetaOffsetUnits=deg  RotationMethod=ArbitraryAxis  RotationAngleUnits=rad  RotationStandardAxis=+Z  RotationAngle=2.0943951023931957  RotationArbitraryAxis=[0.57735026918962573 0.57735026918962562 0.57735026918962573]  FollAlignAxisA=+X  BaseAlignAxisA=+Y  FollAlignAxisB=+Y  BaseAlignAxisB=+Z  RotationSequenceAxes=FollowerAxes  RotationSequence=XYX  RotationSequenceAngles=[0 0 0]  RotationSequenceAnglesUnits=deg  RotationMatrix=[1 0 0; 0 1 0; 0 0 1]
  Transform2 : sm_lib/Frames and Transforms/Rigid Transform  TranslationMethod=Cartesian  TranslationStandardOffset=0  TranslationLengthUnit=mm  TranslationStandardAxis=+Z  TranslationCartesianOffset=[0 0 0]  TranslationROffset=0  TranslationROffsetUnits=m  TranslationZOffset=0  TranslationZOffsetUnits=m  TranslationThetaOffset=0  TranslationThetaOffsetUnits=deg  RotationMethod=AlignedAxes  RotationAngleUnits=deg  RotationStandardAxis=+Z  RotationAngle=90  RotationArbitraryAxis=[-0.57735026918962584 -0.57735026918962562 -0.57735026918962584]  FollAlignAxisA=+Z  BaseAlignAxisA=-Z  FollAlignAxisB=+Y  BaseAlignAxisB=+X  RotationSequenceAxes=FollowerAxes  RotationSequence=XYX  RotationSequenceAngles=[0 0 0]  RotationSequenceAnglesUnits=deg  RotationMatrix=[1 0 0; 0 1 0; 0 0 1]
  Transform3 : sm_lib/Frames and Transforms/Rigid Transform  TranslationMethod=Cartesian  TranslationStandardOffset=0  TranslationLengthUnit=mm  TranslationStandardAxis=+Z  TranslationCartesianOffset=[0 0 0]  TranslationROffset=0  TranslationROffsetUnits=m  TranslationZOffset=0  TranslationZOffsetUnits=m  TranslationThetaOffset=0  TranslationThetaOffsetUnits=deg  RotationMethod=StandardAxis  RotationAngleUnits=deg  RotationStandardAxis=+Z  RotationAngle=180  RotationArbitraryAxis=[-0.57735026918962584 -0.57735026918962562 -0.57735026918962584]  FollAlignAxisA=+Z  BaseAlignAxisA=-Z  FollAlignAxisB=+Y  BaseAlignAxisB=+X  RotationSequenceAxes=FollowerAxes  RotationSequence=XYX  RotationSequenceAngles=[0 0 0]  RotationSequenceAnglesUnits=deg  RotationMatrix=[1 0 0; 0 1 0; 0 0 1]
  Transform4 : sm_lib/Frames and Transforms/Rigid Transform  TranslationMethod=Cartesian  TranslationStandardOffset=0  TranslationLengthUnit=mm  TranslationStandardAxis=+Z  TranslationCartesianOffset=[0 0 0]  TranslationROffset=0  TranslationROffsetUnits=m  TranslationZOffset=0  TranslationZOffsetUnits=m  TranslationThetaOffset=0  TranslationThetaOffsetUnits=deg  RotationMethod=StandardAxis  RotationAngleUnits=deg  RotationStandardAxis=+X  RotationAngle=180  RotationArbitraryAxis=[-0.57735026918962584 -0.57735026918962562 -0.57735026918962584]  FollAlignAxisA=+Z  BaseAlignAxisA=-Z  FollAlignAxisB=+Y  BaseAlignAxisB=+X  RotationSequenceAxes=FollowerAxes  RotationSequence=XYX  RotationSequenceAngles=[0 0 0]  RotationSequenceAnglesUnits=deg  RotationMatrix=[1 0 0; 0 1 0; 0 0 1]
  Transform5 : sm_lib/Frames and Transforms/Rigid Transform  TranslationMethod=Cartesian  TranslationStandardOffset=0  TranslationLengthUnit=mm  TranslationStandardAxis=+Z  TranslationCartesianOffset=[0 0 0]  TranslationROffset=0  TranslationROffsetUnits=m  TranslationZOffset=0  TranslationZOffsetUnits=m  TranslationThetaOffset=0  TranslationThetaOffsetUnits=deg  RotationMethod=StandardAxis  RotationAngleUnits=deg  RotationStandardAxis=+Z  RotationAngle=90  RotationArbitraryAxis=[-0.57735026918962584 -0.57735026918962562 -0.57735026918962584]  FollAlignAxisA=+Z  BaseAlignAxisA=-Z  FollAlignAxisB=+Y  BaseAlignAxisB=+X  RotationSequenceAxes=FollowerAxes  RotationSequence=XYX  RotationSequenceAngles=[0 0 0]  RotationSequenceAnglesUnits=deg  RotationMatrix=[1 0 0; 0 1 0; 0 0 1]
  F : PMIOPort  Side=Left
  F1 : PMIOPort  Port=2  Side=Right
  connections:
  Solid/RConn1 -- ReferenceFrame/RConn1 -- Transform/LConn1 -- Transform1/LConn1
  Transform/RConn1 -- Transform2/LConn1
  Transform1/RConn1 -- Transform4/LConn1
  Transform3/RConn1 -- F/RConn1
  Transform2/RConn1 -- Transform5/LConn1
  Transform4/RConn1 -- F1/RConn1
  Transform5/RConn1 -- Transform3/LConn1

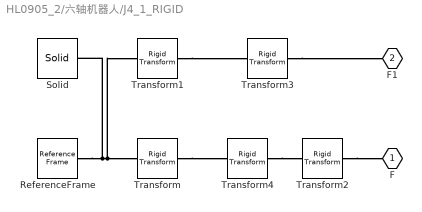
== system HL0905_2/六轴机器人/J4_1_RIGID ==
  ReferenceFrame : sm_lib/Frames and Transforms/Reference Frame
  Solid : sm_lib/Body Elements/Solid  InertiaType=Custom  Mass=5.6600000000000001  MassUnits=kg  CenterOfMass=[-0.27000000000000002 -127.73999999999999 2.2400000000000002]  CenterOfMassUnits=mm  MomentsOfInertia=[57312.889999999999 9191.2999999999993 57306.720000000001]  MomentsOfInertiaUnits=kg*mm^2  ProductsOfInertia=[1680.1400000000001 -5.5199999999999996 95.799999999999997]  ProductsOfInertiaUnits=kg*mm^2  BasedOnType=Density  Density=1000  DensityUnits=kg/(m^3)  DoExposeReferenceFrame=on  SerializedFrames=<Frames/>  GraphicType=FromGeometry  MarkerShape=Sphere  MarkerSize=10  MarkerSizeUnits=m  GraphicVisPropType=SimpleVisualProperties  GraphicDiffuseColor=[1 1 1]  GraphicSpecularColor=[0.5 0.5 0.5 1.0]  GraphicAmbientColor=[0.15 0.15 0.15 1.0]  GraphicEmissiveColor=[0.0 0.0 0.0 1.0]  GraphicShininess=75  GraphicOpacity=1  GeometryShape=FromFile  RectangleSize=[1 1]  RectangleSizeUnits=m  BrickDimensions=[1 1 1]  BrickDimensionUnits=m  CylinderRadius=1  CylinderRadiusUnits=m  CylinderLength=1  CylinderLengthUnits=m  SphereRadius=1  SphereRadiusUnits=m  EllipsoidRadii=[1 1 1]  EllipsoidRadiiUnits=m  ExtrusionCrossSection=[1 1; -1 1; -1 -1; 1 -1]  ExtrusionCrossSectionUnits=m  ExtrusionLength=1  ExtrusionLengthUnits=m  PolygonNumSides=3  PolygonOuterRadius=1  PolygonOuterRadiusUnits=m  ExtGeomFileType=STL  ExtGeomFileName=J4_默认_sldprt.STL  ExtGeomFileUnits=mm  RevolutionCrossSection=[1 1; 1 -1; 2 -1; 2 1]  RevolutionCrossSectionUnits=m  RevolutionExtent=Full  RevolutionAngle=180  RevolutionAngleUnits=deg
  Transform : sm_lib/Frames and Transforms/Rigid Transform  TranslationMethod=Cartesian  TranslationStandardOffset=0  TranslationLengthUnit=mm  TranslationStandardAxis=+Z  TranslationCartesianOffset=[-3.4816594052244909e-13 -31.209572476963913 5.4818372063891729e-12]  TranslationROffset=0  TranslationROffsetUnits=m  TranslationZOffset=0  TranslationZOffsetUnits=m  TranslationThetaOffset=0  TranslationThetaOffsetUnits=deg  RotationMethod=ArbitraryAxis  RotationAngleUnits=rad  RotationStandardAxis=+Z  RotationAngle=2.0943951023932077  RotationArbitraryAxis=[-0.57735026918962995 -0.57735026918962995 -0.5773502691896174]  FollAlignAxisA=+X  BaseAlignAxisA=+Y  FollAlignAxisB=+Y  BaseAlignAxisB=+Z  RotationSequenceAxes=FollowerAxes  RotationSequence=XYX  RotationSequenceAngles=[0 0 0]  RotationSequenceAnglesUnits=deg  RotationMatrix=[1 0 0; 0 1 0; 0 0 1]
  Transform1 : sm_lib/Frames and Transforms/Rigid Transform  TranslationMethod=Cartesian  TranslationStandardOffset=0  TranslationLengthUnit=mm  TranslationStandardAxis=+Z  TranslationCartesianOffset=[1.1102230246251565e-13 -339.99999999999994 -77.256482127756513]  TranslationROffset=0  TranslationROffsetUnits=m  TranslationZOffset=0  TranslationZOffsetUnits=m  TranslationThetaOffset=0  TranslationThetaOffsetUnits=deg  RotationMethod=ArbitraryAxis  RotationAngleUnits=rad  RotationStandardAxis=+Z  RotationAngle=0  RotationArbitraryAxis=[0 0 0]  FollAlignAxisA=+X  BaseAlignAxisA=+Y  FollAlignAxisB=+Y  BaseAlignAxisB=+Z  RotationSequenceAxes=FollowerAxes  RotationSequence=XYX  RotationSequenceAngles=[0 0 0]  RotationSequenceAnglesUnits=deg  RotationMatrix=[1 0 0; 0 1 0; 0 0 1]
  Transform2 : sm_lib/Frames and Transforms/Rigid Transform  TranslationMethod=Cartesian  TranslationStandardOffset=0  TranslationLengthUnit=mm  TranslationStandardAxis=+Z  TranslationCartesianOffset=[0 0 0]  TranslationROffset=0  TranslationROffsetUnits=m  TranslationZOffset=0  TranslationZOffsetUnits=m  TranslationThetaOffset=0  TranslationThetaOffsetUnits=deg  RotationMethod=StandardAxis  RotationAngleUnits=deg  RotationStandardAxis=+Z  RotationAngle=-90  RotationArbitraryAxis=[-0.57735026918962584 -0.57735026918962562 -0.57735026918962584]  FollAlignAxisA=+Z  BaseAlignAxisA=-Z  FollAlignAxisB=+Y  BaseAlignAxisB=+X  RotationSequenceAxes=FollowerAxes  RotationSequence=XYX  RotationSequenceAngles=[0 0 0]  RotationSequenceAnglesUnits=deg  RotationMatrix=[1 0 0; 0 1 0; 0 0 1]
  Transform3 : sm_lib/Frames and Transforms/Rigid Transform  TranslationMethod=Cartesian  TranslationStandardOffset=0  TranslationLengthUnit=mm  TranslationStandardAxis=+Z  TranslationCartesianOffset=[0 0 0]  TranslationROffset=0  TranslationROffsetUnits=m  TranslationZOffset=0  TranslationZOffsetUnits=m  TranslationThetaOffset=0  TranslationThetaOffsetUnits=deg  RotationMethod=StandardAxis  RotationAngleUnits=deg  RotationStandardAxis=+X  RotationAngle=180  RotationArbitraryAxis=[-0.57735026918962584 -0.57735026918962562 -0.57735026918962584]  FollAlignAxisA=+Z  BaseAlignAxisA=-Z  FollAlignAxisB=+Y  BaseAlignAxisB=+X  RotationSequenceAxes=FollowerAxes  RotationSequence=XYX  RotationSequenceAngles=[0 0 0]  RotationSequenceAnglesUnits=deg  RotationMatrix=[1 0 0; 0 1 0; 0 0 1]
  Transform4 : sm_lib/Frames and Transforms/Rigid Transform  TranslationMethod=Cartesian  TranslationStandardOffset=0  TranslationLengthUnit=mm  TranslationStandardAxis=+Z  TranslationCartesianOffset=[0 0 0]  TranslationROffset=0  TranslationROffsetUnits=m  TranslationZOffset=0  TranslationZOffsetUnits=m  TranslationThetaOffset=0  TranslationThetaOffsetUnits=deg  RotationMethod=StandardAxis  RotationAngleUnits=deg  RotationStandardAxis=+X  RotationAngle=180  RotationArbitraryAxis=[-0.57735026918962584 -0.57735026918962562 -0.57735026918962584]  FollAlignAxisA=+Z  BaseAlignAxisA=-Z  FollAlignAxisB=+Y  BaseAlignAxisB=+X  RotationSequenceAxes=FollowerAxes  RotationSequence=XYX  RotationSequenceAngles=[0 0 0]  RotationSequenceAnglesUnits=deg  RotationMatrix=[1 0 0; 0 1 0; 0 0 1]
  F : PMIOPort  Side=Left
  F1 : PMIOPort  Port=2  Side=Right
  connections:
  Solid/RConn1 -- ReferenceFrame/RConn1 -- Transform/LConn1 -- Transform1/LConn1
  Transform4/RConn1 -- Transform2/LConn1
  Transform3/RConn1 -- F1/RConn1
  Transform/RConn1 -- Transform4/LConn1
  Transform2/RConn1 -- F/RConn1
  Transform1/RConn1 -- Transform3/LConn1
